simulink model "Charging_System"  (R2021b)
settings: Solver=FixedStepDiscrete  StartTime=0.0  StopTime=10.0  RelTol=1e-3
undefined symbols (not defined in the file): Ion, Lithium
libraries: spsSeriesRLCBranchLib x3, spsBatteryLib x1, spsBuckConverterLib x1, spsCurrentMeasurementLib x1, spsGroundLib x1, spsPVArrayLib x1, eePwmGenerator x1, spspowerguiLib x1
settings Model: Creator=KennyBoum-biha  LastModifiedBy=KennyBoum-biha

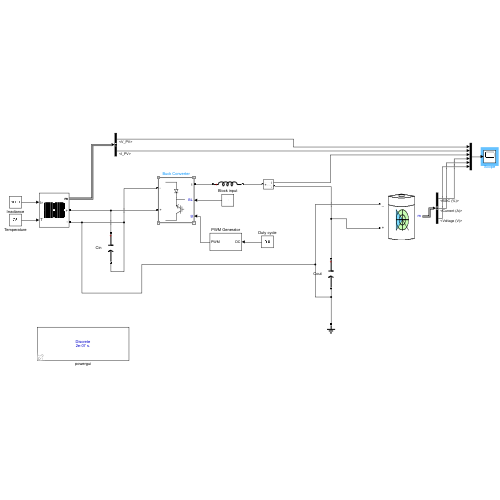
[thumbnail: Simulink's stored preview of the top-level diagram]
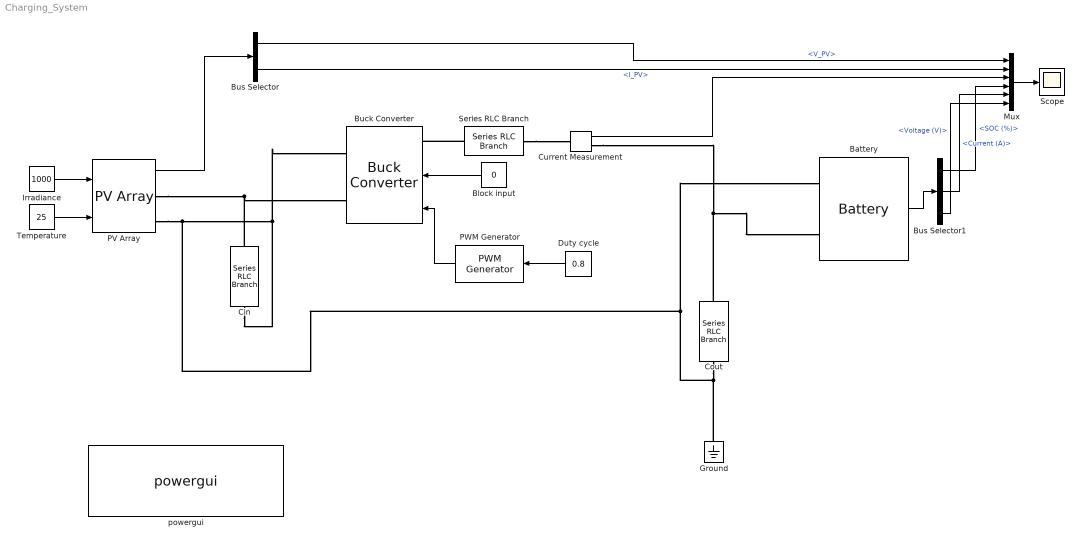
== system Charging_System ==
  Battery : spsBatteryLib/Battery  BatType=Lithium-Ion  ShowTempParam=off  ThermalPreset=no  ShowAgeParam=off  NomV=48  NomQ=0.5  SOC=50  Batt_Tr=5  PresetModel=on  MaxQ=0.5  MinV=36  FullV=55.8714  Dis_rate=0.21739  R=0.96  Normal_OP=0.45217  expZone="[51.8585    0.0245652]"  current=[6.5 13 32.5]  Units=Time  Tci=20  NomT=20  T2=-30  MaxQ2=4.8  FullV2=7.1  Normal_OP2=5.655  expZone2="[6.58           1]"  Rca=0.6  ti=2000  Dp=0  Neq0=0  Tsim=1e6  Ta1=25  Qeol=5.4*0.9  Reol=0.013333*1.2  Char_age=[2.3478, 3]  Dis_age=[2.3478, 10]  N1=1500  N2=10500  N3=1000  N4=1400  Ta2=45  N5=950
  Block input : Constant  Value=0
  Buck Converter : spsBuckConverterLib/Buck Converter  ModelType=Switching devices  Ron=1e-3  Rs=1e6  Cs=inf  Vforward=[0,0]  Ron_Diode=1e-3  Rs_Diode=1e6  Cs_Diode=inf  Vf_Diode=1e-3  Rs_CurrentSource=inf
      settings: SourceProductBaseCode=PS
  Bus Selector : BusSelector  OutputSignals=V_PV,I_PV
  Bus Selector1 : BusSelector  OutputSignals=SOC (%),Current (A),Voltage (V)
  Cin : spsSeriesRLCBranchLib/Series RLC Branch  LConnTagsString=__new0  RConnTagsString=__new0  BranchType=C  Resistance=1  Inductance=47e-6  SetiL0=off  InitialCurrent=0  Capacitance=100e-6  Setx0=off  InitialVoltage=0  Measurements=None
  Cout : spsSeriesRLCBranchLib/Series RLC Branch  LConnTagsString=__new0  RConnTagsString=__new0  BranchType=C  Resistance=1  Inductance=47e-6  SetiL0=off  InitialCurrent=0  Capacitance=100e-6  Setx0=off  InitialVoltage=0  Measurements=None
  Current Measurement : spsCurrentMeasurementLib/Current Measurement  PhasorSimulation=off  OutputType=Complex  PSBequivalent=0
  Duty cycle : Constant  Value=0.8
  Ground : spsGroundLib/Ground  LConnTagsString=a
  Irradiance : Constant  Value=1000
  Mux : Mux  Inputs=6
  PV Array : spsPVArrayLib/PV Array  Npar=1  Nser=2  PlotType=array @ 1000 W/m2 & specified temperatures  S_vec="[ 1000  500  100 ]"  Temp_C_vec="[ 45 25  ]"  ModuleName=User-defined  PlotWhenSelected=off  Pm=213.15  Ncell=60  Voc=36.3  Isc=7.84  Vm=29  Im=7.35  beta_Voc_pc=-0.36099  alpha_Isc_pc=0.102  beta_Voc=-0.13104  alpha_Isc=0.0079968  IL=7.8654  I0=2.9273e-10  nI=0.98119  Rsh=313.0553  Rs=0.39381  RobustModel=off  RobustCellTemperature=313.3991  BAL=on  Tc=1e-6  Tfilter=5e-5
  PWM Generator : eePwmGenerator/PWM Generator  CarrCount=Up  Tper=0.001  Tdelay=0  Ts=2e-7
  Scope : Scope
  Series RLC Branch : spsSeriesRLCBranchLib/Series RLC Branch  LConnTagsString=__new0  RConnTagsString=__new0  BranchType=L  Resistance=1  Inductance=47e-6  SetiL0=off  InitialCurrent=0  Capacitance=1e-6  Setx0=off  InitialVoltage=0  Measurements=None
  Temperature : Constant  Value=25
  powergui : spspowerguiLib/powergui  Priority=1  SimulationMode=Discrete  SampleTime=2e-7  frequency=60  Iterations=50  frequencyindice=0  Pbase=100e6  ErrMax=1e-4  UnitsV=kV  UnitsW=MW  buscounter=0  FunctionMessages=off  echomessages=off  EnableUseOfTLC=off  CurrentSourceSwitches=off  DisableSnubberDevices=off  DisableRonSwitches=off  DisableVfSwitches=off  DisplayEquations=off  AutomaticDiscreteSolvers=off  SolverType=Tustin/Backward Euler (TBE)  Interpol=off  ExternalGateDelay=off  methode=off  Ts=100  x0status=blocks  SPID=on  SwTol=0  HookPort=off  NonlinearTolerance=1e-4  nMaxIteration=100  ContinueOnMaxIteration=off  RestoreLinks=warning  ResistiveCurrentMeasurement=off  Frange=[0:2:500]  Ylog=off  Xlog=on  ShowGrid=off  save=off  variable=ZData  structure=0  ZoomFFT=off  StartTime=0.0  cycles=1  DisplayStyle=1  fundamental=60  FreqAxis=off  MaxFrequency=1000  frequencyindicesteady=1  RmsSteady=1  display=off
  wires:
  Irradiance/1 -> PV Array/1
  Temperature/1 -> PV Array/2
  PWM Generator/1 -> Buck Converter/1
  Block input/1 -> Buck Converter/2
  Current Measurement/1 -> Mux/3
  Duty cycle/1 -> PWM Generator/1
  Mux/1 -> Scope/1
  Battery/1 -> Bus Selector1/1
  PV Array/1 -> Bus Selector/1
  Bus Selector/1 -> Mux/1  "<V_PV>"
  Bus Selector/2 -> Mux/2  "<I_PV>"
  Bus Selector1/1 -> Mux/4  "<SOC (%)>"
  Bus Selector1/2 -> Mux/5  "<Current (A)>"
  Bus Selector1/3 -> Mux/6  "<Voltage (V)>"
  connections:
  PV Array/RConn1 -- Buck Converter/RConn1 -- Cin/LConn1
  Ground/LConn1 -- Cin/RConn1 -- Buck Converter/RConn2 -- PV Array/RConn2 -- Battery/LConn2 -- Cout/RConn1
  Series RLC Branch/LConn1 -- Buck Converter/LConn1
  Series RLC Branch/RConn1 -- Current Measurement/LConn1
  Current Measurement/RConn1 -- Cout/LConn1 -- Battery/LConn1
